simulink model "kinodynamic_plant"  (R2026b)
settings: Solver=ode4  FixedStep=0.001
undefined symbols (not defined in the file): plantInitialState
settings Model: DataDictionary=vehicle_control.sldd  Creator=rayyu  LastModifiedBy=bxr240009
settings ModelReferenceCC: ModelReferenceMinAlgLoopOccurrences=on
settings RTWCC: GPUComputeCapability=5.0
settings GRTTargetCC: CombineOutputUpdateFcns=off

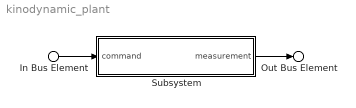
== system kinodynamic_plant ==
  In Bus Element : Inport  PortName=u
  Subsystem : Subsystem
  Out Bus Element : Outport  PortName=y
  wires:
  In Bus Element/1 -> Subsystem/1(command)
  Subsystem/1(measurement) -> Out Bus Element/1

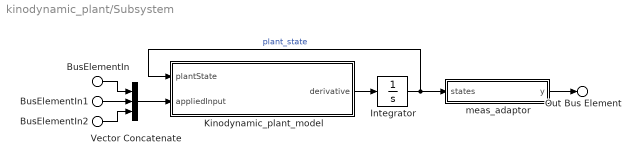
== system kinodynamic_plant/Subsystem ==
  BusElementIn : Inport  PortName=command  Element=Fx
  BusElementIn1 : Inport  PortName=command  Element=Fy
  BusElementIn2 : Inport  PortName=command  Element=Mz
  Integrator : Integrator  InitialCondition=plantInitialState
  Kinodynamic_plant_model : MATLAB Function  TreatAsAtomicUnit=on
  Vector Concatenate : Concatenate  NumInputs=3
  meas_adaptor : Subsystem
  Out Bus Element : Outport  PortName=measurement
  wires:
  Kinodynamic_plant_model/1(derivative) -> Integrator/1
  meas_adaptor/1(y) -> Out Bus Element/1
  Integrator/1 -> Kinodynamic_plant_model/1(plantState), meas_adaptor/1(states)  "plant_state"
  BusElementIn/1 -> Vector Concatenate/1
  BusElementIn1/1 -> Vector Concatenate/2
  BusElementIn2/1 -> Vector Concatenate/3
  Vector Concatenate/1 -> Kinodynamic_plant_model/2(appliedInput)

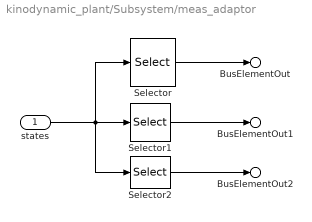
== system kinodynamic_plant/Subsystem/meas_adaptor ==
  states : Inport
  Selector : Selector  InputPortWidth=7  IndexOptions=Index vector (dialog)  Indices=[1 2 3 4 5]  OutputSizes=1  RuntimeRangeChecks=off
  Selector1 : Selector  InputPortWidth=7  IndexOptions=Index vector (dialog)  Indices=6  OutputSizes=1  RuntimeRangeChecks=off
  Selector2 : Selector  InputPortWidth=7  IndexOptions=Index vector (dialog)  Indices=7  OutputSizes=1  RuntimeRangeChecks=off
  BusElementOut : Outport  PortName=y  Element=x
  BusElementOut1 : Outport  PortName=y  Element=vx
  BusElementOut2 : Outport  PortName=y  Element=s
  wires:
  states/1 -> Selector/1, Selector2/1, Selector1/1
  Selector/1 -> BusElementOut/1
  Selector1/1 -> BusElementOut1/1
  Selector2/1 -> BusElementOut2/1

== matlab function kinodynamic_plant/Subsystem/Kinodynamic_plant_model ==
  data: plantState input size=[7 1]; derivative output size=[7 1]; appliedInput input size=[3 1]; plantContext parameter
function derivative = evaluatePlant(plantState, appliedInput, plantContext)
%EVALUATEPLANT Evaluate the shared seven-state plant equations.
%
% plantState   : [e; psi; v; vy; gamma; vx; s]
% appliedInput : [Fx; Fy; Mz]

derivative = ecu.model.plant_rhs( ...
    plantState, appliedInput, plantContext);

end
